simulink model "sens_imu_model"  (R2026b)
settings: Solver=VariableStepAuto
values from neighbouring files (symbols this model uses):
  D = zeros(nx, ny, 'uint8')    [sens_lidar2d_fast.m]
  P = (P + P.')/2    [sens_nav_ekf.m]
undefined symbols (not defined in the file or in its folder): fractalcoef, Ts
libraries: simulink x5, sharedutil x3, mspsensorlib x1, robotcorelib x1
settings Model: Creator=aomar  LastModifiedBy=aomar

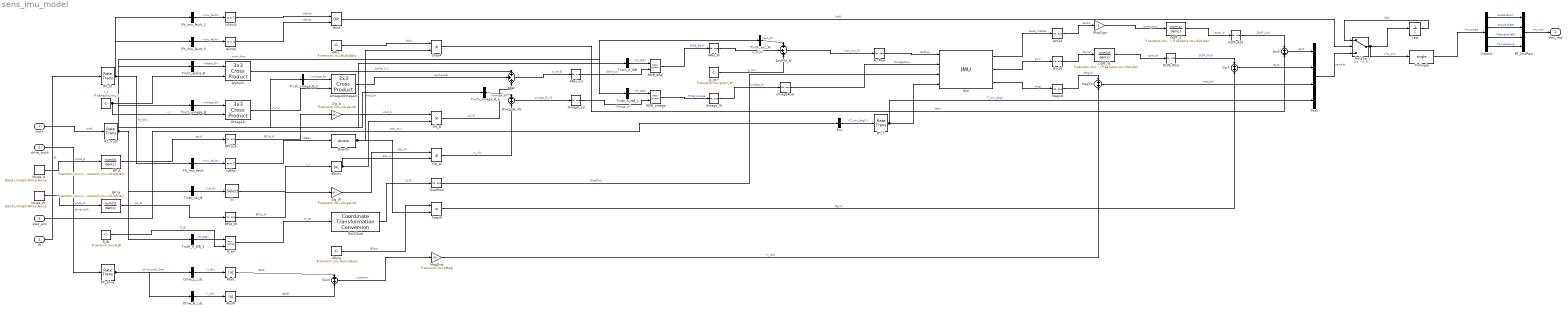
== system sens_imu_model ==
  truth : Inport  OutDataTypeStr=Bus: Bus_TruthState  SampleTime=Ts.base
  drive_truth : Inport  Port=2  OutDataTypeStr=Bus: Bus_DriveTruth  SampleTime=Ts.base
  elec_env : Inport  Port=3  OutDataTypeStr=Bus: Bus_ElecEnv  SampleTime=Ts.hk
  flt : Inport  Port=4  OutDataTypeStr=Bus: Bus_FaultInject  SampleTime=Ts.ctrl
  ARel : Sum  Inputs=+++
  ARel_W : Reshape
  ARel_col : Reshape  OutputDimensionality=Column vector (2-D)
  AbsIL : Abs  SaturateOnIntegerOverflow=off
  AbsIR : Abs  SaturateOnIntegerOverflow=off
  AbsVx : Abs  SaturateOnIntegerOverflow=off
  Acc1d : Reshape
  AccF : Sum
  AccIMU_W : Sum  Inputs=+++
  AccRow : Reshape  OutputDimensionality=Row vector (2-D)
  AlphaXr : sharedutil/3x3 Cross Product  aMode=aMode
      settings: LibrarySourceBlock=aerolibutil/3x3 Cross Product
  BC_ImuRaw : BusCreator  Inputs=4  OutDataTypeStr=Bus: Bus_ImuRaw  NonVirtualBus=on
      settings: InheritFromInputs=off
  BP1d_A : Reshape
  BP1d_W : Reshape
  BP_A : DiscreteTransferFcn  Numerator=P.sensors.imu.vib.bpNum  Denominator=P.sensors.imu.vib.bpDen  SampleTime=Ts.imu
  BP_W : DiscreteTransferFcn  Numerator=P.sensors.imu.vib.bpNum  Denominator=P.sensors.imu.vib.bpDen  SampleTime=Ts.imu
  BiasOn : DataTypeConversion  OutDataTypeStr=double  RndMeth=Nearest  SaturateOnIntegerOverflow=off
  DLPF_A : DiscreteTransferFcn  Numerator=P.sensors.imu.dlpf.num  Denominator=P.sensors.imu.dlpf.den  SampleTime=Ts.imu
  DLPF_A1d : Reshape
  DLPF_W : DiscreteTransferFcn  Numerator=P.sensors.imu.dlpf.num  Denominator=P.sensors.imu.dlpf.den  SampleTime=Ts.imu
  DLPF_W1d : Reshape
  Drive_L_i_dc : BusSelector  OutputSignals=L.i_dc
  Drive_R_i_dc : BusSelector  OutputSignals=R.i_dc
  Env : BusSelector  OutputSignals=T_imu_degC
  Flt_imu_fault : BusSelector  OutputSignals=imu_fault
  Flt_imu_fault_2 : BusSelector  OutputSignals=imu_fault
  Flt_imu_fault_3 : BusSelector  OutputSignals=imu_fault
  Gyr1d : Reshape
  GyrF : Sum
  Hold : Logic  Operator=OR  AllPortsSameDT=off  OutDataTypeStr=boolean
  HoldSw : Switch  Criteria=u2 ~= 0  SaturateOnIntegerOverflow=off  InputSameDT=off
  IMU : mspsensorlib/IMU  DispRefFrame=ENU  TemperaturePort=on  Temperature=25  MagneticFieldPort=off  MagneticFieldNED=[ 27.5550, -2.4169, -16.0849 ]  MagneticFieldENU=P.sensors.imu.magENU  SeedDouble=P.sensors.imu.seed  SimulateUsing=Code generation  AccelParamsMeasurementRange=P.sensors.imu.accel.MeasurementRange  AccelParamsResolution=P.sensors.imu.accel.Resolution  AccelParamsConstantBias=-P.sensors.imu.accel.ConstantBias  AccelParamsAxesMisalignment=P.sensors.imu.accel.AxesMisalignment  AccelParamsNoiseDensity=P.sensors.imu.accel.NoiseDensity  AccelParamsBiasInstability=P.sensors.imu.accel.BiasInstability  AccelParamsBiasInstabilityNumerator=fractalcoef().Numerator  AccelParamsBiasInstabilityDenominator=fractalcoef().Denominator  AccelParamsRandomWalk=P.sensors.imu.accel.RandomWalk  AccelParamsNoiseType=double-sided  AccelParamsTemperatureBias=-P.sensors.imu.accel.TemperatureBias  AccelParamsTemperatureScaleFactor=P.sensors.imu.accel.TemperatureScaleFactor  GyroParamsMeasurementRange=P.sensors.imu.gyro.MeasurementRange  GyroParamsResolution=P.sensors.imu.gyro.Resolution  GyroParamsConstantBias=P.sensors.imu.gyro.ConstantBias  GyroParamsAxesMisalignment=P.sensors.imu.gyro.AxesMisalignment  GyroParamsAccelerationBias=P.sensors.imu.gyro.AccelerationBias  GyroParamsNoiseDensity=P.sensors.imu.gyro.NoiseDensity  GyroParamsBiasInstability=P.sensors.imu.gyro.BiasInstability  GyroParamsBiasInstabilityNumerator=fractalcoef().Numerator  GyroParamsBiasInstabilityDenominator=fractalcoef().Denominator  GyroParamsRandomWalk=P.sensors.imu.gyro.RandomWalk  GyroParamsNoiseType=double-sided  GyroParamsTemperatureBias=P.sensors.imu.gyro.TemperatureBias  GyroParamsTemperatureScaleFactor=P.sensors.imu.gyro.TemperatureScaleFactor  MagParamsMeasurementRange=P.sensors.imu.mag.MeasurementRange  MagParamsResolution=P.sensors.imu.mag.Resolution  MagParamsConstantBias=P.sensors.imu.mag.ConstantBias  MagParamsAxesMisalignment=[ 100, 0, 0; 0, 100, 0; 0, 0, 100 ]  MagParamsNoiseDensity=P.sensors.imu.mag.NoiseDensity  MagParamsBiasInstability=P.sensors.imu.mag.BiasInstability  MagParamsBiasInstabilityNumerator=fractalcoef().Numerator  MagParamsBiasInstabilityDenominator=fractalcoef().Denominator  MagParamsRandomWalk=[ 0, 0, 0 ]  MagParamsNoiseType=double-sided  MagParamsTemperatureBias=P.sensors.imu.mag.TemperatureBias  MagParamsTemperatureScaleFactor=[ 0, 0, 0 ]
  ISum : Sum
  IsBias : simulink/Logic and Bit Operations/Compare To Constant  relop===  const=2  OutDataTypeStr=boolean
  IsDrop : simulink/Logic and Bit Operations/Compare To Constant  relop===  const=3  OutDataTypeStr=boolean
  IsStuck : simulink/Logic and Bit Operations/Compare To Constant  relop===  const=1  OutDataTypeStr=boolean
  Last : UnitDelay  InitialCondition=zeros(10,1)  SampleTime=Ts.imu
  Mag1d : Reshape
  MagDist : Gain  Gain=P.sensors.imu.kMagI
  MagTot : Sum
  Noise_A : simulink/Sources/Band-Limited White Noise  Cov=P.sensors.imu.vib.cov*[1 1 1]  Ts=Ts.imu  seed=P.sensors.imu.vib.seedA
  Noise_W : simulink/Sources/Band-Limited White Noise  Cov=P.sensors.imu.vib.cov*[1 1 1]  Ts=Ts.imu  seed=P.sensors.imu.vib.seedW
  OmegaB_vib : Sum
  OmegaRow : Reshape  OutputDimensionality=Row vector (2-D)
  OmegaXOmegaXr : sharedutil/3x3 Cross Product  aMode=aMode
      settings: LibrarySourceBlock=aerolibutil/3x3 Cross Product
  OmegaXr : sharedutil/3x3 Cross Product  aMode=aMode
      settings: LibrarySourceBlock=aerolibutil/3x3 Cross Product
  Omega_W : Reshape
  Omega_col : Reshape  OutputDimensionality=Column vector (2-D)
  Pack : Mux  Inputs=[3 3 3 1]
  PhysSign : Gain  Gain=-1
  QuatRow : Reshape  OutputDimensionality=Row vector (2-D)
  RT_T : RateTransition  OutPortSampleTime=Ts.imu
  RT_drive : RateTransition  OutPortSampleTime=Ts.imu
  RT_flt : RateTransition  OutPortSampleTime=Ts.imu
  RT_truth : RateTransition  OutPortSampleTime=Ts.imu
  RWB_aRel : Product  Multiplication=Matrix(*)
  RWB_omega : Product  Multiplication=Matrix(*)
  R_BI : Constant  Value=P.sensors.imu.R_BI
  R_WI : Product  Multiplication=Matrix(*)
  Rot2Quat : robotcorelib/Coordinate Transformation Conversion  InputRepresentation=Rotation Matrix  InputEulerSequence=ZYX  ShowTrVecInputPort=on  OutputRepresentation=Quaternion  OutputEulerSequence=ZYX  ShowTrVecOutputPort=on  SimulateUsing=Code generation
      settings: LibrarySourceBlock=navlib/Utilities/Coordinate Transformation Conversion
  Sig_A : Gain  Gain=P.sensors.imu.vib.gainA
  Sig_W : Gain  Gain=P.sensors.imu.vib.gainW
  StepA : Product  Inputs=**
  StepW : Product  Inputs=**
  ToSingle : DataTypeConversion  OutDataTypeStr=single  RndMeth=Nearest  SaturateOnIntegerOverflow=off
  Truth_R_WB : BusSelector  OutputSignals=R_WB
  Truth_R_WB_2 : BusSelector  OutputSignals=R_WB
  Truth_R_WB_3 : BusSelector  OutputSignals=R_WB
  Truth_acc_W : BusSelector  OutputSignals=acc_W
  Truth_alpha_B : BusSelector  OutputSignals=alpha_B
  Truth_omega_B : BusSelector  OutputSignals=omega_B
  Truth_omega_B_2 : BusSelector  OutputSignals=omega_B
  Truth_omega_B_3 : BusSelector  OutputSignals=omega_B
  Truth_vel_B : BusSelector  OutputSignals=vel_B
  Unpack : Demux  Outputs=[3 3 3 1]
  Vib_A : Product  Inputs=**
  Vib_W : Product  Inputs=**
  Vx : Selector  InputPortWidth=3  IndexOptions=Index vector (dialog)  Indices=1  OutputSizes=1
  dAcc : Constant  Value=P.sensors.imu.fault.dAcc
  dGyro : Constant  Value=P.sensors.imu.fault.dGyro
  g_corr : Constant  Value=P.sensors.imu.gcorr_W
  r_I : Constant  Value=P.sensors.imu.r
  imu_raw : Outport  OutDataTypeStr=Bus: Bus_ImuRaw
  wires:
  truth/1 -> RT_truth/1  "truth"
  drive_truth/1 -> RT_drive/1  "drive_truth"
  Noise_A/1 -> BP_A/1  "white_A"
  Noise_W/1 -> BP_W/1  "white_W"
  elec_env/1 -> Env/1  "elec_env"
  flt/1 -> RT_flt/1  "flt"
  r_I/1 -> AlphaXr/2, OmegaXr/2  "r_I"
  R_BI/1 -> R_WI/2  "R_BI"
  RT_flt/1 -> Flt_imu_fault/1, Flt_imu_fault_2/1, Flt_imu_fault_3/1  "flt_5ms"
  RT_drive/1 -> Drive_R_i_dc/1, Drive_L_i_dc/1  "drive_truth_5ms"
  RT_truth/1 -> Truth_R_WB_3/1, Truth_acc_W/1, Truth_R_WB/1, Truth_alpha_B/1, Truth_vel_B/1, Truth_omega_B_2/1, Truth_omega_B_3/1, Truth_R_WB_2/1, Truth_omega_B/1  "truth_5ms"
  BP_A/1 -> BP1d_A/1  "bp_A"
  BP_W/1 -> BP1d_W/1  "bp_W"
  Flt_imu_fault_2/1 -> IsStuck/1  "<imu_fault>"
  Flt_imu_fault_3/1 -> IsDrop/1  "<imu_fault>"
  Truth_alpha_B/1 -> AlphaXr/1  "<alpha_B>"
  Truth_omega_B/1 -> OmegaXr/1  "<omega_B>"
  Flt_imu_fault/1 -> IsBias/1  "<imu_fault>"
  Truth_vel_B/1 -> Vx/1  "<vel_B>"
  Truth_R_WB_3/1 -> R_WI/1  "<R_WB>"
  Drive_L_i_dc/1 -> AbsIL/1  "<i_dc>"
  Drive_R_i_dc/1 -> AbsIR/1  "<i_dc>"
  IsStuck/1 -> Hold/1  "IsStuck"
  IsDrop/1 -> Hold/2  "IsDrop"
  BP1d_A/1 -> Sig_A/1  "BP1d_A"
  IsBias/1 -> BiasOn/1  "IsBias"
  BP1d_W/1 -> Sig_W/1  "BP1d_W"
  R_WI/1 -> Rot2Quat/1  "R_WI"
  AbsIL/1 -> ISum/1  "AbsIL"
  AbsIR/1 -> ISum/2  "AbsIR"
  Vx/1 -> AbsVx/1  "v_x"
  AlphaXr/1 -> ARel/1  "alpha_x_r"
  OmegaXr/1 -> OmegaXOmegaXr/2  "w_x_r"
  Truth_omega_B_2/1 -> OmegaXOmegaXr/1  "<omega_B>"
  ISum/1 -> MagDist/1  "i_traction"
  Hold/1 -> HoldSw/2  "hold"
  dAcc/1 -> StepA/1  "dAcc"
  Sig_A/1 -> Vib_A/1  "vib1_A"
  AbsVx/1 -> Vib_A/2, Vib_W/2  "abs_vx"
  Sig_W/1 -> Vib_W/1  "vib1_W"
  dGyro/1 -> StepW/1  "dGyro"
  OmegaXOmegaXr/1 -> ARel/2  "centripetal"
  BiasOn/1 -> StepA/2, StepW/2  "bias_on"
  Rot2Quat/1 -> QuatRow/1  "q_WI"
  StepA/1 -> AccF/2  "dacc"
  Vib_W/1 -> OmegaB_vib/2  "w_vib"
  QuatRow/1 -> IMU/3  "QuatRow"
  StepW/1 -> GyrF/2  "dgyro"
  MagDist/1 -> MagTot/2  "m_dist"
  ARel/1 -> ARel_col/1  "a_rel_B"
  OmegaB_vib/1 -> Omega_col/1  "omega_B_vib"
  ARel_col/1 -> RWB_aRel/2  "ARel_col"
  Omega_col/1 -> RWB_omega/2  "Omega_col"
  Truth_R_WB/1 -> RWB_aRel/1  "<R_WB>"
  Truth_R_WB_2/1 -> RWB_omega/1  "<R_WB>"
  RWB_aRel/1 -> ARel_W/1  "RWB_aRel"
  RWB_omega/1 -> Omega_W/1  "RWB_omega"
  ARel_W/1 -> AccIMU_W/2  "a_rel_W"
  g_corr/1 -> AccIMU_W/3  "g_corr"
  Omega_W/1 -> OmegaRow/1  "omega_W"
  Truth_acc_W/1 -> AccIMU_W/1  "<acc_W>"
  AccIMU_W/1 -> AccRow/1  "acc_imu_W"
  OmegaRow/1 -> IMU/2  "OmegaRow"
  Env/1 -> RT_T/1  "<T_imu_degC>"
  AccRow/1 -> IMU/1  "AccRow"
  RT_T/1 -> IMU/4, Pack/4  "T_imu_degC"
  IMU/1 -> Acc1d/1  "accel_matlab"
  IMU/2 -> Gyr1d/1  "gyro"
  IMU/3 -> Mag1d/1  "mag"
  Acc1d/1 -> PhysSign/1  "Acc1d"
  Gyr1d/1 -> DLPF_W/1  "Gyr1d"
  Mag1d/1 -> MagTot/1  "Mag1d"
  MagTot/1 -> Pack/3  "mag_tot"
  PhysSign/1 -> DLPF_A/1  "accel_phys"
  DLPF_W/1 -> DLPF_W1d/1  "gyro_lp"
  DLPF_W1d/1 -> GyrF/1  "DLPF_W1d"
  DLPF_A/1 -> DLPF_A1d/1  "accel_lp"
  GyrF/1 -> Pack/2  "GyrF"
  DLPF_A1d/1 -> AccF/1  "DLPF_A1d"
  AccF/1 -> Pack/1  "AccF"
  Pack/1 -> HoldSw/3  "sample"
  HoldSw/1 -> Last/1, ToSingle/1  "imu_out"
  Last/1 -> HoldSw/1  "last"
  ToSingle/1 -> Unpack/1  "imu_single"
  Unpack/1 -> BC_ImuRaw/1  "Acceleration"
  Unpack/2 -> BC_ImuRaw/2  "AngularRate"
  Unpack/3 -> BC_ImuRaw/3  "MagneticField"
  Unpack/4 -> BC_ImuRaw/4  "Temperature"
  BC_ImuRaw/1 -> imu_raw/1  "imu_raw"
  Vib_A/1 -> ARel/3  "a_vib"
  Truth_omega_B_3/1 -> OmegaB_vib/1  "<omega_B>"
